simulink model "AS2308_MIL_Baseline_v3"  (R2023b)
settings: Solver=ode4  StartTime=0.0  StopTime=10.0  FixedStep=ts  RelTol=1e-3
values from neighbouring files (symbols this model uses):
  Kas = Kis/Kps    (= 17.76)    [AS2308_calculate_pi_control_cc.m]
  Kis = a*Kps    (= 2.04192887437)    [AS2308_calculate_pi_control_cc.m]
  Kps = w_cs/b    (= 0.114973472656)    [AS2308_calculate_pi_control_cc.m]
  Vdc = 12    [AS2308_calculate_pi_control_cc.m]
undefined symbols (not defined in the file or in its folder): SpeedRef_cmd
settings Model: Creator=kimdaeyoung  LastModifiedBy=kimdaeyoung

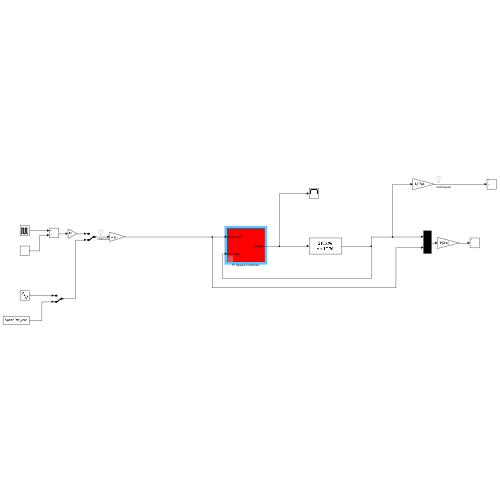
[thumbnail: Simulink's stored preview of the top-level diagram]
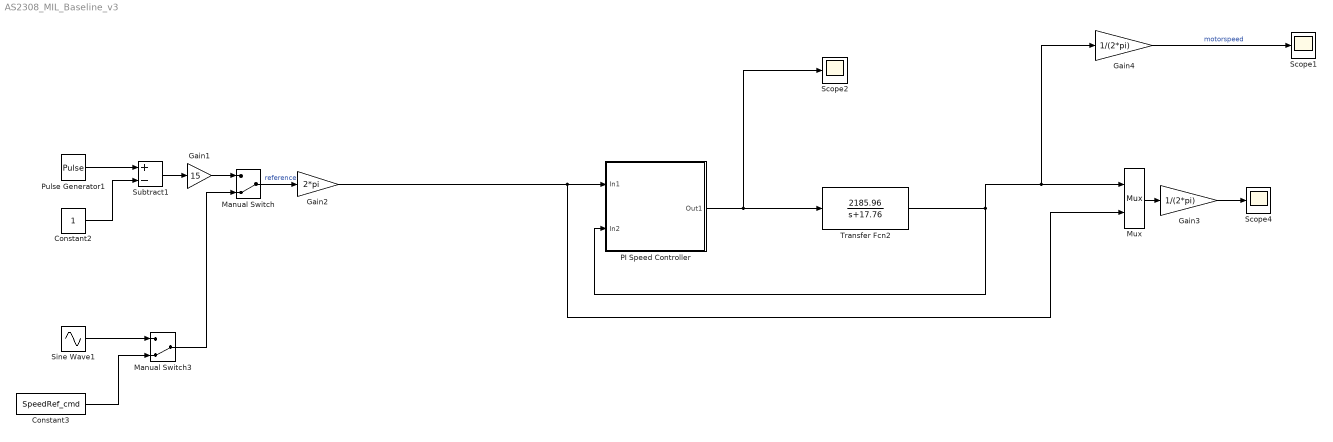
== system AS2308_MIL_Baseline_v3 ==
  Constant2 : Constant
  Constant3 : Constant  Value=SpeedRef_cmd
  Gain1 : Gain  Gain=15
  Gain2 : Gain  Gain=2*pi
  Gain3 : Gain  Gain=1/(2*pi)
  Gain4 : Gain  Gain=1/(2*pi)
  Manual Switch : ManualSwitch  CurrentSetting=0
  Manual Switch3 : ManualSwitch  CurrentSetting=0
  Mux : Mux  Inputs=2
  PI Speed Controller : Subsystem
      mask DialogControl ParameterGroupVar Prompt: 파라미터
      mask Display:
      | % Red background
      | patch([0 100 100 0], [0 0 100 100], [1 0 0]);
      | 
      | % Port labels
      | port_label('input', 1, 'Speed ref');
      | port_label('input', 2, 'dot theta');
      | port_label('output', 1, 'voltage');
      | 
      | % Block name
  Pulse Generator1 : DiscretePulseGenerator  PulseType=Time based  Amplitude=2  PulseWidth=50
  Scope1 : Scope
  Scope2 : Scope
  Scope4 : Scope
  Sine Wave1 : Sin  Amplitude=15  Frequency=15  SampleTime=0
  Subtract1 : Sum  Inputs=+-
  Transfer Fcn2 : TransferFcn  Numerator=[2185.96]  Denominator=[1 17.76]
  wires:
  Manual Switch3/1 -> Manual Switch/2
  PI Speed Controller/1(Out1) -> Transfer Fcn2/1, Scope2/1
  Gain3/1 -> Scope4/1
  Constant3/1 -> Manual Switch3/2
  Mux/1 -> Gain3/1
  Sine Wave1/1 -> Manual Switch3/1
  Constant2/1 -> Subtract1/2
  Pulse Generator1/1 -> Subtract1/1
  Gain4/1 -> Scope1/1  "motorspeed"
  Gain2/1 -> Mux/2, PI Speed Controller/1(In1)
  Subtract1/1 -> Gain1/1
  Manual Switch/1 -> Gain2/1  "reference"
  Gain1/1 -> Manual Switch/1
  Transfer Fcn2/1 -> Gain4/1, Mux/1, PI Speed Controller/2(In2)

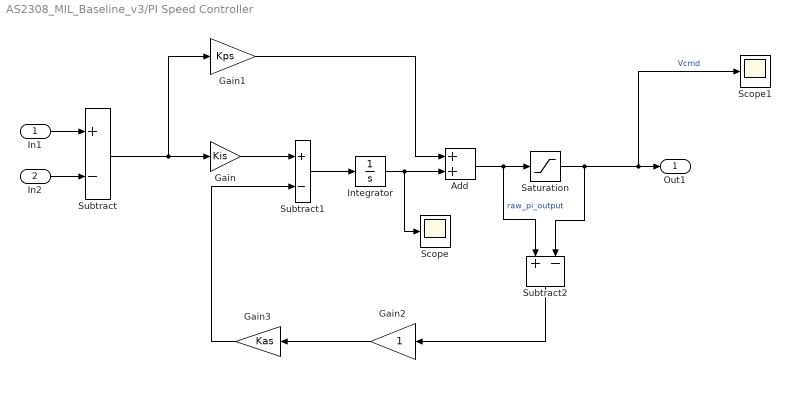
== system AS2308_MIL_Baseline_v3/PI Speed Controller ==
  In1 : Inport
  In2 : Inport  Port=2
  Add : Sum
  Gain : Gain  Gain=Kis
  Gain1 : Gain  Gain=Kps
  Gain2 : Gain
  Gain3 : Gain  Gain=Kas
  Integrator : Integrator
  Saturation : Saturate  UpperLimit=Vdc  LowerLimit=-Vdc
  Scope : Scope
  Scope1 : Scope
  Subtract : Sum  Inputs=+-
  Subtract1 : Sum  Inputs=+-
  Subtract2 : Sum  Inputs=+-
  Out1 : Outport
  wires:
  Subtract/1 -> Gain1/1, Gain/1
  Gain/1 -> Subtract1/1
  Subtract1/1 -> Integrator/1
  Integrator/1 -> Scope/1, Add/2
  Gain1/1 -> Add/1
  In1/1 -> Subtract/1
  In2/1 -> Subtract/2
  Add/1 -> Subtract2/1, Saturation/1  "raw_pi_output"
  Saturation/1 -> Scope1/1, Out1/1, Subtract2/2  "Vcmd"
  Subtract2/1 -> Gain2/1
  Gain2/1 -> Gain3/1
  Gain3/1 -> Subtract1/2
